simulink library "DiscretePID"  (R2026a)
settings: Solver=VariableStepAuto
undefined symbols (not defined in the file): pidCfg
settings Model: Creator=24322  LastModifiedBy=24322

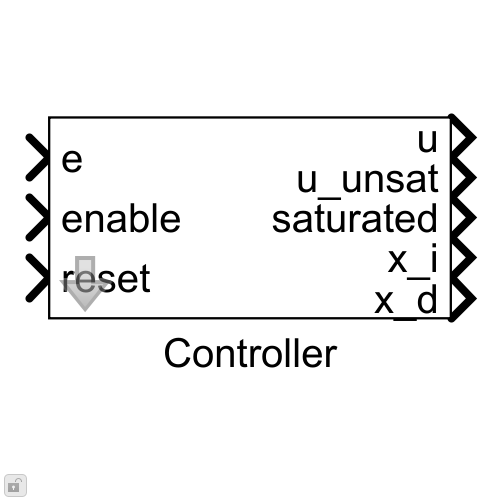
[thumbnail: Simulink's stored preview of the top-level diagram]
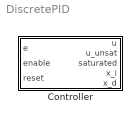
== system DiscretePID ==
  Controller : Subsystem  mask{Kp=pidCfg.Kp, Ki=pidCfg.Ki, Ts=pidCfg.Ts, UMin=pidCfg.UMin, UMax=pidCfg.UMax, X0=pidCfg.X0, Kaw=pidCfg.Kaw, Kd=pidCfg.Kd, Tf=pidCfg.Tf}
      mask Display:
      | port_label('input',1,'e');
      | port_label('input',2,'enable');
      | port_label('input',3,'reset');
      | port_label('output',1,'u');
      | port_label('output',2,'u_unsat');
      | port_label('output',3,'saturated');
      | port_label('output',4,'x_i');
      | port_label('output',5,'x_d');

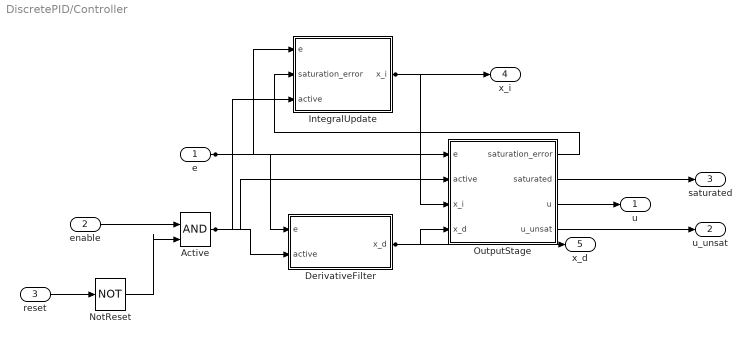
== system DiscretePID/Controller ==
  e : Inport
  enable : Inport  Port=2  OutDataTypeStr=boolean
  reset : Inport  Port=3  OutDataTypeStr=boolean
  Active : Logic  IconShape=distinctive  AllPortsSameDT=off  OutDataTypeStr=boolean
  DerivativeFilter : Subsystem
  IntegralUpdate : Subsystem
  NotReset : Logic  Operator=NOT  Inputs=1  IconShape=distinctive  AllPortsSameDT=off  OutDataTypeStr=boolean
  OutputStage : Subsystem
  u : Outport
  u_unsat : Outport  Port=2
  saturated : Outport  Port=3
  x_i : Outport  Port=4
  x_d : Outport  Port=5
  wires:
  DerivativeFilter/1(x_d) -> x_d/1, OutputStage/4(x_d)
  reset/1 -> NotReset/1
  OutputStage/1(saturation_error) -> IntegralUpdate/2(saturation_error)
  IntegralUpdate/1(x_i) -> OutputStage/3(x_i), x_i/1
  OutputStage/4(u_unsat) -> u_unsat/1
  OutputStage/3(u) -> u/1
  OutputStage/2(saturated) -> saturated/1
  Active/1 -> OutputStage/2(active), IntegralUpdate/3(active), DerivativeFilter/2(active)
  NotReset/1 -> Active/2
  enable/1 -> Active/1
  e/1 -> IntegralUpdate/1(e), OutputStage/1(e), DerivativeFilter/1(e)

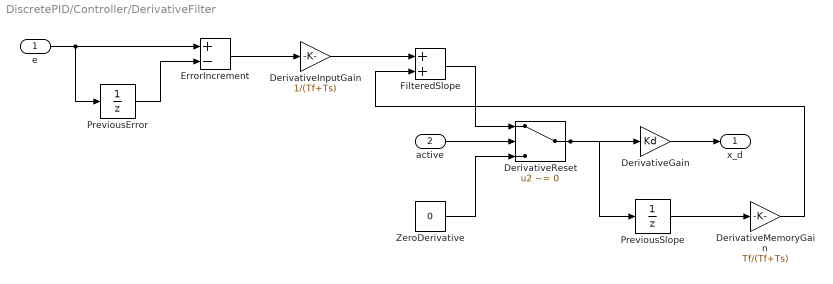
== system DiscretePID/Controller/DerivativeFilter ==
  e : Inport
  active : Inport  Port=2
  DerivativeGain : Gain  Gain=Kd
  DerivativeInputGain : Gain  Gain=1/(Tf+Ts)
  DerivativeMemoryGain : Gain  Gain=Tf/(Tf+Ts)
  DerivativeReset : Switch  Criteria=u2 ~= 0  SaturateOnIntegerOverflow=off  InputSameDT=off
  ErrorIncrement : Sum  Inputs=+-
  FilteredSlope : Sum
  PreviousError : UnitDelay  SampleTime=Ts
  PreviousSlope : UnitDelay  SampleTime=Ts
  ZeroDerivative : Constant  Value=0
  x_d : Outport
  wires:
  ZeroDerivative/1 -> DerivativeReset/3
  active/1 -> DerivativeReset/2
  FilteredSlope/1 -> DerivativeReset/1
  DerivativeMemoryGain/1 -> FilteredSlope/2
  DerivativeInputGain/1 -> FilteredSlope/1
  PreviousSlope/1 -> DerivativeMemoryGain/1
  ErrorIncrement/1 -> DerivativeInputGain/1
  PreviousError/1 -> ErrorIncrement/2
  e/1 -> PreviousError/1, ErrorIncrement/1
  DerivativeGain/1 -> x_d/1
  DerivativeReset/1 -> DerivativeGain/1, PreviousSlope/1

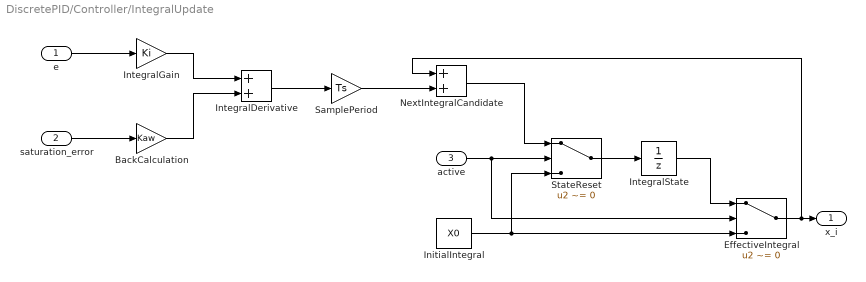
== system DiscretePID/Controller/IntegralUpdate ==
  e : Inport
  saturation_error : Inport  Port=2
  active : Inport  Port=3
  BackCalculation : Gain  Gain=Kaw
  EffectiveIntegral : Switch  Criteria=u2 ~= 0  SaturateOnIntegerOverflow=off  InputSameDT=off
  InitialIntegral : Constant  Value=X0
  IntegralDerivative : Sum
  IntegralGain : Gain  Gain=Ki
  IntegralState : UnitDelay  InitialCondition=X0  SampleTime=Ts
  NextIntegralCandidate : Sum
  SamplePeriod : Gain  Gain=Ts
  StateReset : Switch  Criteria=u2 ~= 0  SaturateOnIntegerOverflow=off  InputSameDT=off
  x_i : Outport
  wires:
  EffectiveIntegral/1 -> x_i/1, NextIntegralCandidate/1
  IntegralDerivative/1 -> SamplePeriod/1
  NextIntegralCandidate/1 -> StateReset/1
  InitialIntegral/1 -> EffectiveIntegral/3, StateReset/3
  StateReset/1 -> IntegralState/1
  IntegralState/1 -> EffectiveIntegral/1
  BackCalculation/1 -> IntegralDerivative/2
  IntegralGain/1 -> IntegralDerivative/1
  SamplePeriod/1 -> NextIntegralCandidate/2
  saturation_error/1 -> BackCalculation/1
  e/1 -> IntegralGain/1
  active/1 -> EffectiveIntegral/2, StateReset/2

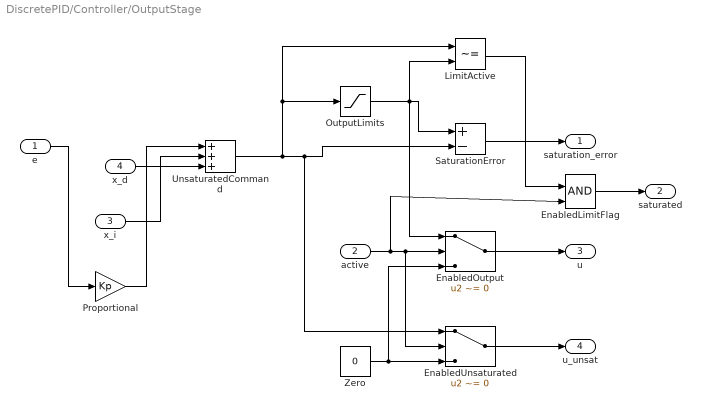
== system DiscretePID/Controller/OutputStage ==
  e : Inport
  active : Inport  Port=2
  x_i : Inport  Port=3
  x_d : Inport  Port=4
  EnabledLimitFlag : Logic  IconShape=distinctive  AllPortsSameDT=off  OutDataTypeStr=boolean
  EnabledOutput : Switch  Criteria=u2 ~= 0  SaturateOnIntegerOverflow=off  InputSameDT=off
  EnabledUnsaturated : Switch  Criteria=u2 ~= 0  SaturateOnIntegerOverflow=off  InputSameDT=off
  LimitActive : RelationalOperator  Operator=~=  OutDataTypeStr=boolean  RndMeth=Simplest  InputSameDT=off
  OutputLimits : Saturate  UpperLimit=UMax  LowerLimit=UMin
  Proportional : Gain  Gain=Kp
  SaturationError : Sum  Inputs=+-
  UnsaturatedCommand : Sum  Inputs=+++
  Zero : Constant  Value=0
  saturation_error : Outport
  saturated : Outport  Port=2
  u : Outport  Port=3
  u_unsat : Outport  Port=4
  wires:
  UnsaturatedCommand/1 -> SaturationError/2, EnabledUnsaturated/1, OutputLimits/1, LimitActive/1
  LimitActive/1 -> EnabledLimitFlag/1
  OutputLimits/1 -> SaturationError/1, EnabledOutput/1, LimitActive/2
  Zero/1 -> EnabledUnsaturated/3, EnabledOutput/3
  EnabledOutput/1 -> u/1
  EnabledUnsaturated/1 -> u_unsat/1
  EnabledLimitFlag/1 -> saturated/1
  x_i/1 -> UnsaturatedCommand/2
  SaturationError/1 -> saturation_error/1
  active/1 -> EnabledOutput/2, EnabledUnsaturated/2, EnabledLimitFlag/2
  x_d/1 -> UnsaturatedCommand/3
  Proportional/1 -> UnsaturatedCommand/1
  e/1 -> Proportional/1
